simulink model "slexPrinterExample"  (R2025b)
settings: Solver=FixedStepDiscrete  StartTime=0.0  StopTime=200  RelTol=1e-3  EnableMultiTasking=on
model workspace (MATLAB code in the model file):
  | INK_MIN=1;
  | PRINT_RATE=1;
undefined symbols (not defined in the file or in its folder): job, queuePrintJob
settings Model: ModifiedByFormat=The MathWorks Inc.  ExtModeAutoUpdateStatusClock=off  Creator=The MathWorks, Inc.  LastModifiedBy=The MathWorks Inc.
settings SolverCC: AlgebraicLoopSolver=TrustRegion
settings DataIOCC: LimitDataPoints=on  SaveFormat=Array  SignalLoggingName=sigsOut
settings OptimizationCC: ReuseModelBlockBuffer=off  ExpressionDepthLimit=2147483647.0  InitFltsAndDblsToZero=on  EfficientMapNaN2IntZero=off  LifeSpan=Inf  EfficientTunableParamExpr=on
settings DebuggingCC: SaveWithParameterizedLinksMsg=none  SignalResolutionControl=TryResolveAllWithWarning  BlockPriorityViolationMsg=error  UnconnectedInputMsg=warning  UnconnectedOutputMsg=warning  UnconnectedLineMsg=warning  AllowSymbolicDim=off  StateNameClashWarn=warning  PregeneratedLibrarySubsystemCodeDiagnostic=none  SFUnexpectedBacktrackingDiag=warning  SFNoUnconditionalDefaultTransitionDiag=warning  SFExecutionAtInitializationDiag=none  ArithmeticOperatorsInVariantConditions=warning
settings HardwareCC: ProdBitPerPointer=32.0  ProdBitPerSizeT=32.0  ProdBitPerPtrDiffT=32.0  ProdLargestAtomicFloat=None  ProdIntDivRoundTo=Undefined  ProdEndianess=Unspecified  ProdWordSize=32.0  ProdHWDeviceType=32-bit Generic  TargetBitPerPointer=64.0  TargetBitPerSizeT=64.0  TargetBitPerPtrDiffT=64.0  TargetLongLongMode=on  TargetIntDivRoundTo=Zero  TargetEndianess=LittleEndian  TargetWordSize=64.0  TargetHWDeviceType=MATLAB Host  ProdEqTarget=off
settings ModelReferenceCC: EnableRefExpFcnMdlSchedulingChecks=on  PropagateSignalLabelsOutOfModel=off
settings SFSimCC: SFSimEcho=off  SimIntegrity=off  SimUseLocalCustomCode=off  SimParseCustomCode=off  MATLABDynamicMemAlloc=off  CustomCodeUndefinedFunction=UseInterfaceOnly
settings RTWCC: SystemTargetFile=ert.tlc  TemplateMakefile=ert_default_tmf  GenerateReport=on  RTWUseLocalCustomCode=off  IncludeHyperlinkInReport=on  LaunchReport=on  GenerateTraceInfo=on  GenerateTraceReport=on  GenerateTraceReportSl=on  GenerateTraceReportSf=on  GenerateTraceReportEml=on  GPUComputeCapability=3.5  DLArmComputeVersion=19.05  Description=Real-Time Workshop Embedded Coder
settings CodeAppCC: IgnoreCustomStorageClasses=off  CustomSymbolStrType=$N$R$M  StateflowObjectComments=on  InternalIdentifier=Classic
settings ERTTargetCC: InlinedParameterPlacement=Hierarchical  ERTCustomFileTemplate=example_file_process.tlc  ConvertIfToSwitch=off  SuppressUnreachableDefaultCases=off  MultiwordLength=2048.0  GenerateSampleERTMain=on
settings ConfigComp: CovMetricSettings=dcmtr  CovSaveCumulativeToWorkspaceVar=on  CovSaveSingleToWorkspaceVar=on  CovExternalEMLEnable=off  CovSFcnEnable=off

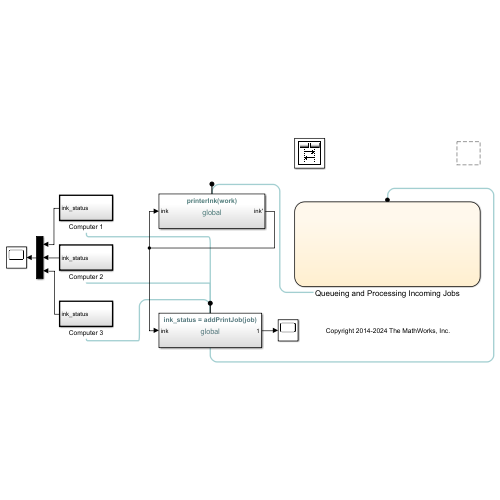
[thumbnail: Simulink's stored preview of the top-level diagram]
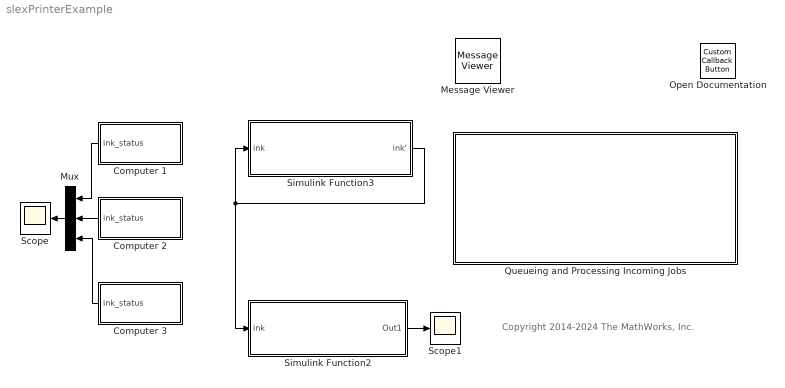
== system slexPrinterExample ==
  note: Copyright 2014-2024 The MathWorks, Inc.
  Computer 1 : Subsystem  TreatAsAtomicUnit=on
  Computer 2 : Subsystem  TreatAsAtomicUnit=on
  Computer 3 : Subsystem  TreatAsAtomicUnit=on
  Message Viewer : MessageViewer  SavedRootId=#
  Mux : Mux  Inputs=3
  Open Documentation : CustomCallbackButton  Configuration="{\"components\":[{\"name\":\"BackgroundImageComponent\",\"settings\":{\"image\":{\"size\":[0,0],\"src\":\"default\",\"srcOrientation\":\"Right\"},\"position\":[0,0,1,1]}},{\"name\":\"ButtonStateComponent\",\"settings\":{\"buttonType\":\"momentary\",\"clickFcn\":\"showExample('stateflow\\/ShareFcnsAcrossSLandSFExample')\",\"onValue\":1,\"position\":[0,0,1,1],\"pressDelay\":\"500\",\"pressFcn\":\"\",\"repeatInterval\":\"0\",\"states\":[{\"horizontalAlignment\":\"center\",\"image\":{\"position\":[0,0,1,1],\"src\":\"default\",\"srcOrientation\":\"Right\"},\"label\":{\"color\":[0.01176470588,0.01176470588,0.01176470588,1],\"icon\":{\"size\":[0,0],\"src\":\"default\",\"srcOrientation\":\"Right\"},\"iconPlacement\":\"left\",\"text\":{\"content\":\"?\"}},\"labelOffset\":[0,0],\"verticalAlignment\":\"middle\"},{\"horizontalAlignment\":\"center\",\"image\":{\"position\":[0,0,1,1],\"src\":\"default\",\"srcOrientation\":\"Right\"},\"label\":{\"color\":[0.01176470588,0.01176470588,0.01176470588,1],\"icon\":{\"size\":[0,0],\"src\":\"default\",\"srcOrientation\":\"Right\"},\"iconPlacement\":\"left\",\"text\":{\"content\":\"?\"}},\"labelOffset\":[0,0],\"verticalAlignment\":\"middle\"},{\"horizontalAlignment\":\"center\",\"image\":{\"position\":[0,0,1,1],\"src\":\"default\",\"srcOrientation\":\"Right\"},\"label\":{\"color\":[0.01176470588,0.01176470588,0.01176470588,1],\"icon\":{\"size\":[0,0],\"src\":\"default\",\"srcOrientation\":\"Right\"},\"iconPlacement\":\"left\",\"text\":{\"content\":\"?\"}},\"labelOffset\":[0,0],\"verticalAlignment\":\"middle\"},{\"horizontalAlignment\":\"center\",\"image\":{\"position\":[0,0,1,1],\"src\":\"default\",\"srcOrientation\":\"Right\"},\"label\":{\"color\":[0.01176470588,0.01176470588,0.01176470588,1],\"icon\":{\"size\":[0,0],\"src\":\"default\",\"srcOrientation\":\"Right\"},\"iconPlacement\":\"left\",\"text\":{\"content\":\"?\"}},\"labelOffset\":[0,0],\"verticalAlignment\":\"middle\"}]}},{\"name\":\"ForegroundImageComponent\",\"settings\":{\"image\":{\"size\":[0,0],\"src\":\"default\",\"srcOrientation\":\"Right\"},\"isForeground\":1,\"position\":[0,0,1,1]}}],\"settings\":{\"BindingType\":\"standalone\",\"backgroundColor\":[244,244,244,1],\"backgroundOffset\":0.2,\"backgroundOpacity\":1,\"fixedAspectRatio\":\"off\",\"foregroundColor\":[0.01176470588,0.01176470588,0.01176470588,1],\"migratedFromLegacy\":true,\"useBackgroundColor\":true,\"variant\":\"callback\",\"version\":\"R2023a\"},\"type\":\"Button\"}"  CustomBackgroundColor="{\"color\":[0.9568627451,0.9568627451,0.9568627451],\"show\":true}"
      settings: OpenFcn=showExample('simulink_features/MonitoringInkStatusOnASharedPrinterExample')
  Queueing and Processing Incoming Jobs : Stateflow chart  TreatAsAtomicUnit=on
  Scope : Scope
      settings: DataLoggingSaveFormat=Array
  Scope1 : Scope
      settings: DataLoggingSaveFormat=Array
  Simulink Function2 : Subsystem  TreatAsAtomicUnit=on
  Simulink Function3 : Subsystem  TreatAsAtomicUnit=on
  wires:
  Simulink Function3/1(ink') -> Simulink Function2/1(ink), Simulink Function3/1(ink)
  Computer 1/1(ink_status) -> Mux/1
  Computer 2/1(ink_status) -> Mux/2
  Computer 3/1(ink_status) -> Mux/3
  Mux/1 -> Scope/1
  Simulink Function2/1(Out1) -> Scope1/1

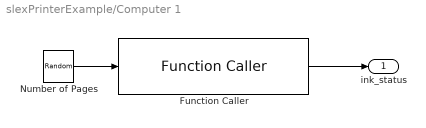
== system slexPrinterExample/Computer 1 ==
  Function Caller : FunctionCaller  FunctionPrototype=ink_status = addPrintJob(job)  InputArgumentSpecifications=<Enter example>  OutputArgumentSpecifications=<Enter example>
  Number of Pages : UniformRandomNumber  Minimum=0  Maximum=.5  SampleTime=1
  ink_status : Outport  VectorParamsAs1DForOutWhenUnconnected=off
  wires:
  Number of Pages/1 -> Function Caller/1
  Function Caller/1 -> ink_status/1

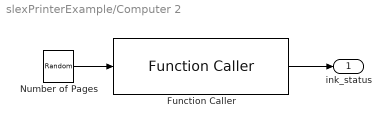
== system slexPrinterExample/Computer 2 ==
  Function Caller : FunctionCaller  FunctionPrototype=ink_status = addPrintJob(job)  InputArgumentSpecifications=<Enter example>  OutputArgumentSpecifications=<Enter example>
  Number of Pages : UniformRandomNumber  Minimum=0  Maximum=.5  SampleTime=1
  ink_status : Outport  InitialOutput=100  VectorParamsAs1DForOutWhenUnconnected=off
  wires:
  Number of Pages/1 -> Function Caller/1
  Function Caller/1 -> ink_status/1

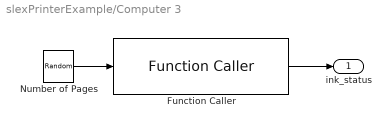
== system slexPrinterExample/Computer 3 ==
  Function Caller : FunctionCaller  FunctionPrototype=ink_status = addPrintJob(job)  InputArgumentSpecifications=<Enter example>  OutputArgumentSpecifications=<Enter example>
  Number of Pages : UniformRandomNumber  Minimum=0  Maximum=.5  SampleTime=1
  ink_status : Outport  InitialOutput=100  VectorParamsAs1DForOutWhenUnconnected=off
  wires:
  Number of Pages/1 -> Function Caller/1
  Function Caller/1 -> ink_status/1

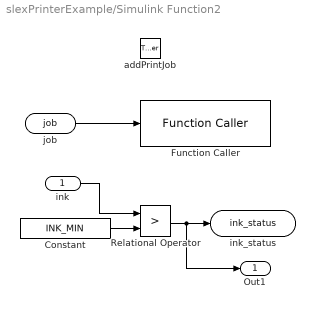
== system slexPrinterExample/Simulink Function2 ==
  ink : Inport
      settings: LatchInputForFeedbackSignals=on
  addPrintJob : TriggerPort  TriggerType=function-call  IsSimulinkFunction=on  FunctionName=addPrintJob  VariantControl=Variant
  Constant : Constant  Value=INK_MIN
  Function Caller : FunctionCaller  FunctionPrototype=queuePrintJob(job)  InputArgumentSpecifications=1  OutputArgumentSpecifications=<Enter example>
  Relational Operator : RelationalOperator  Operator=>  OutDataTypeStr=boolean  InputSameDT=off
  job : ArgIn  DisableCoverage=on  ArgumentName=job
  ink_status : ArgOut  OutDataTypeStr=boolean  ArgumentName=ink_status
  Out1 : Outport  VectorParamsAs1DForOutWhenUnconnected=off
  wires:
  job/1 -> Function Caller/1
  ink/1 -> Relational Operator/1
  Constant/1 -> Relational Operator/2
  Relational Operator/1 -> Out1/1, ink_status/1

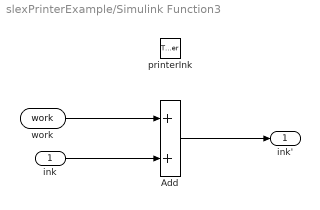
== system slexPrinterExample/Simulink Function3 ==
  ink : Inport
      settings: LatchInputForFeedbackSignals=on
  printerInk : TriggerPort  TriggerType=function-call  IsSimulinkFunction=on  FunctionName=printerInk  VariantControl=Variant
  Add : Sum
  work : ArgIn  DisableCoverage=on  ArgumentName=work
  ink' : Outport  InitialOutput=100  VectorParamsAs1DForOutWhenUnconnected=off
  wires:
  work/1 -> Add/1
  Add/1 -> ink'/1
  ink/1 -> Add/2

== stateflow chart slexPrinterExample/Queueing and Processing Incoming Jobs ==
  settings: updateMethod=DISCRETE  sampleTime=1
  state Idle
  state queuePrintJob(job) [function]
    (default) -> (junction 1905) : { work = work + job; }
  state Busy
    du:
    work = work-PRINT_RATE;
    printerInk(-PRINT_RATE);
  (default) -> Idle
  Idle -> Busy : [work > 0]
  Busy -> Idle : [work <= 0]
  data: job function_input double size=1; work local double; PRINT_RATE parameter
